simulink model "FrameBlendTest"  (R2026b)
settings: Solver=FixedStepDiscrete  StopTime=blendTestCfg.Duration  FixedStep=blendTestCfg.Ts
PostLoadFcn:
  | addpath(fullfile(fileparts(get_param(bdroot,'FileName')),'..','build_process'));initialize_frame_blend_test(bdroot);
model workspace (MAT data in the model file):
  blendTestCfg.Ts = 5e-05
  blendTestCfg.Inputs = [1  0  0  2  0  0  0  1  0; 1  0  0  2  0  0  1  1  0; 1  0  0  2  1.57079632679  0  0  1  0; 1  0  0  2  0  1.57079632679  0  1  0; 2  -1  -1  3  3.12  -3.1  0.4  1  0; 2  -1  -1  3  0.7  -0.2  -1  1  0; 2  -1  -1  3  0.7  -0.2  2  1  0; 2  -1  -1  3  0.7  -0.2  0.4  0  0; 2  -1  -1  3  0.7  -0.2  0.4  1  1; 0  0  0  0  1.2  -1.6  0.5  1  0; 3  4  -4  3  1  -2  0.5  1  0; 2  -1  -1  3  31.8159265359  0.4  0  1  0; -2  1  1  -3  3.14159265359  0  0.3  1  0]
  blendTestCfg.Duration = 0.0006
  testStim.time = [0; 5e-05; 0.0001; 0.00015; 0.0002; 0.00025; 0.0003; 0.00035; 0.0004; 0.00045; 0.0005; 0.00055; 0.0006]
  testStim.signals.values = [1  0  0  2  0  0  0  1  0; 1  0  0  2  0  0  1  1  0; 1  0  0  2  1.57079632679  0  0  1  0; 1  0  0  2  0  1.57079632679  0  1  0; 2  -1  -1  3  3.12  -3.1  0.4  1  0; 2  -1  -1  3  0.7  -0.2  -1  1  0; 2  -1  -1  3  0.7  -0.2  2  1  0; 2  -1  -1  3  0.7  -0.2  0.4  0  0; 2  -1  -1  3  0.7  -0.2  0.4  1  1; 0  0  0  0  1.2  -1.6  0.5  1  0; 3  4  -4  3  1  -2  0.5  1  0; 2  -1  -1  3  31.8159265359  0.4  0  1  0; -2  1  1  -3  3.14159265359  0  0.3  1  0]
  testStim.signals.dimensions = 9
libraries: ClarkePark x1
settings Model: Creator=24322  LastModifiedBy=24322

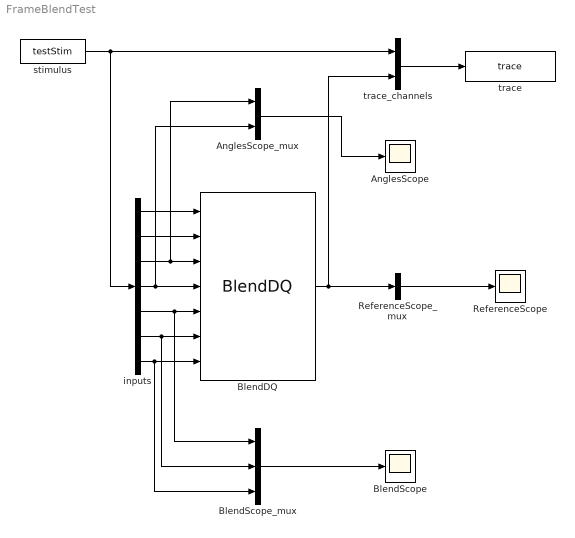
== system FrameBlendTest ==
  AnglesScope : Scope
  AnglesScope_mux : Mux  Inputs=2
  BlendDQ : ClarkePark/BlendDQ  SystemSampleTime=-1  VariantActivationTime=update diagram  EmptyChoice=off  PassThrough=off  PassThroughVariantControl=(default)  EmptyChoiceVariantControl=(default)  AllowFlexibleInterface=on  Latency=0  AutoFrameSizeCalculation=off
  BlendScope : Scope
  BlendScope_mux : Mux  Inputs=3
  ReferenceScope : Scope
  ReferenceScope_mux : Mux  Inputs=1
  inputs : Demux  Outputs=[2 2 1 1 1 1 1]
  stimulus : FromWorkspace  VariableName=testStim  SampleTime=blendTestCfg.Ts  Interpolate=off  OutputAfterFinalValue=Holding final value
  trace : ToWorkspace  VariableName=trace  SaveFormat=Structure With Time  SampleTime=-1
  trace_channels : Mux  Inputs=2
  wires:
  BlendScope_mux/1 -> BlendScope/1
  AnglesScope_mux/1 -> AnglesScope/1
  ReferenceScope_mux/1 -> ReferenceScope/1
  inputs/7 -> BlendDQ/7, BlendScope_mux/3
  inputs/6 -> BlendDQ/6, BlendScope_mux/2
  inputs/5 -> BlendDQ/5, BlendScope_mux/1
  inputs/4 -> AnglesScope_mux/2, BlendDQ/4
  inputs/3 -> BlendDQ/3, AnglesScope_mux/1
  inputs/2 -> BlendDQ/2
  inputs/1 -> BlendDQ/1
  trace_channels/1 -> trace/1
  BlendDQ/1 -> trace_channels/2, ReferenceScope_mux/1
  stimulus/1 -> inputs/1, trace_channels/1
